simulink model "PV_BESS_EMS_PRICE"  (R2026a)
settings: Solver=FixedStepDiscrete  StopTime=86400  FixedStep=900
undefined symbols (not defined in the file): E_batt_kWh, P_batt_max_kW, P_grid_limit_kW, precharge_enable, price_aware_enable, price_low_threshold_RMB_MWh
settings Model: Creator=陈进  LastModifiedBy=陈进

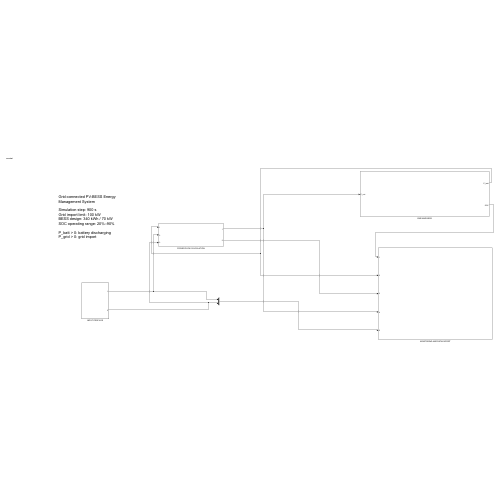
[thumbnail: Simulink's stored preview of the top-level diagram]
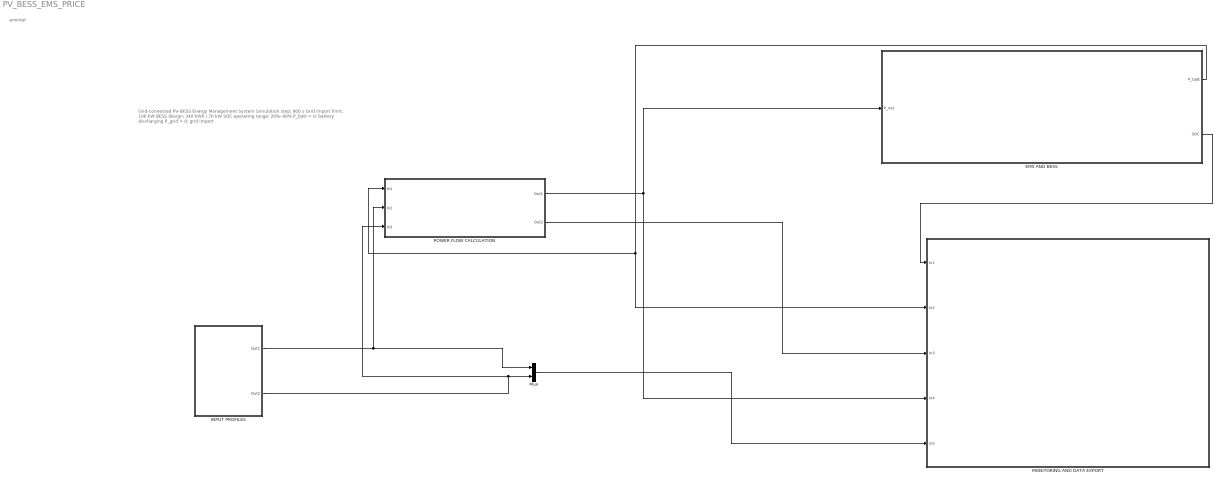
== system PV_BESS_EMS_PRICE ==
  note: Grid-connected PV-BESS Energy Management System
      |
      | Simulation step: 900 s
      | Grid import limit: 100 kW
      | BESS design: 340 kWh / 70 kW
      | SOC operating range: 20%–90%
      |
      | P_batt > 0: battery discharging
      | P_grid > 0: grid import
  note: annotat
  EMS AND BESS : Subsystem
  INPUT PROFILES : Subsystem
  MONITORING AND DATA EXPORT : Subsystem
  Mux : Mux  Inputs=2
  POWER FLOW CALCULATION : Subsystem
  wires:
  INPUT PROFILES/2(Out2) -> POWER FLOW CALCULATION/3(In3), Mux/2
  INPUT PROFILES/1(Out1) -> Mux/1, POWER FLOW CALCULATION/2(In2)
  POWER FLOW CALCULATION/1(Out1) -> MONITORING AND DATA EXPORT/4(In4), EMS AND BESS/1(P_net)
  EMS AND BESS/1(P_batt) -> POWER FLOW CALCULATION/1(In1), MONITORING AND DATA EXPORT/2(In2)
  EMS AND BESS/2(SOC) -> MONITORING AND DATA EXPORT/1(In1)
  POWER FLOW CALCULATION/2(Out2) -> MONITORING AND DATA EXPORT/3(In3)
  Mux/1 -> MONITORING AND DATA EXPORT/5(In5)

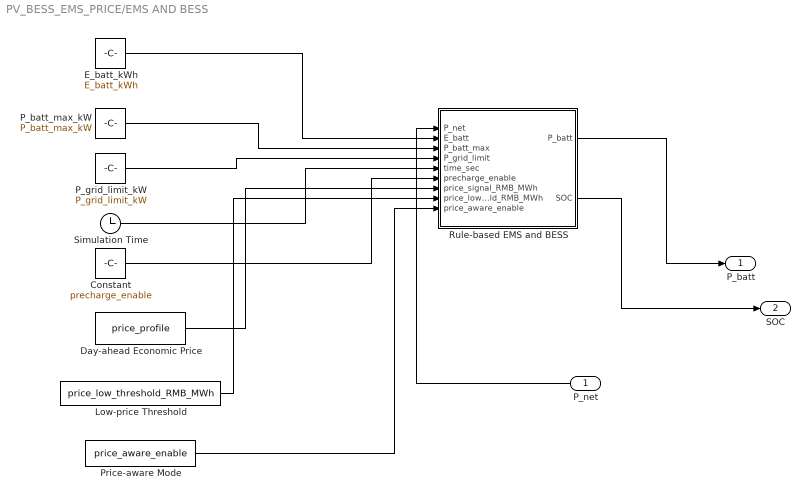
== system PV_BESS_EMS_PRICE/EMS AND BESS ==
  P_net : Inport
  Constant : Constant  Value=precharge_enable
  Day-ahead Economic Price : FromWorkspace  VariableName=price_profile
  E_batt_kWh : Constant  Value=E_batt_kWh
  Low-price Threshold : Constant  Value=price_low_threshold_RMB_MWh
  P_batt_max_kW : Constant  Value=P_batt_max_kW
  P_grid_limit_kW : Constant  Value=P_grid_limit_kW
  Price-aware Mode : Constant  Value=price_aware_enable
  Rule-based EMS and BESS : MATLAB Function  TreatAsAtomicUnit=on
  Simulation Time : Clock
  P_batt : Outport
  SOC : Outport  Port=2
  wires:
  E_batt_kWh/1 -> Rule-based EMS and BESS/2(E_batt)
  Rule-based EMS and BESS/1(P_batt) -> P_batt/1
  P_batt_max_kW/1 -> Rule-based EMS and BESS/3(P_batt_max)
  Rule-based EMS and BESS/2(SOC) -> SOC/1
  P_net/1 -> Rule-based EMS and BESS/1(P_net)
  Simulation Time/1 -> Rule-based EMS and BESS/5(time_sec)
  Constant/1 -> Rule-based EMS and BESS/6(precharge_enable)
  P_grid_limit_kW/1 -> Rule-based EMS and BESS/4(P_grid_limit)
  Day-ahead Economic Price/1 -> Rule-based EMS and BESS/7(price_signal_RMB_MWh)
  Low-price Threshold/1 -> Rule-based EMS and BESS/8(price_low_threshold_RMB_MWh)
  Price-aware Mode/1 -> Rule-based EMS and BESS/9(price_aware_enable)

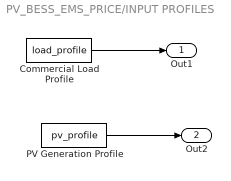
== system PV_BESS_EMS_PRICE/INPUT PROFILES ==
  Commercial Load Profile : FromWorkspace  VariableName=load_profile
  PV Generation Profile : FromWorkspace  VariableName=pv_profile
  Out1 : Outport
  Out2 : Outport  Port=2
  wires:
  PV Generation Profile/1 -> Out2/1
  Commercial Load Profile/1 -> Out1/1

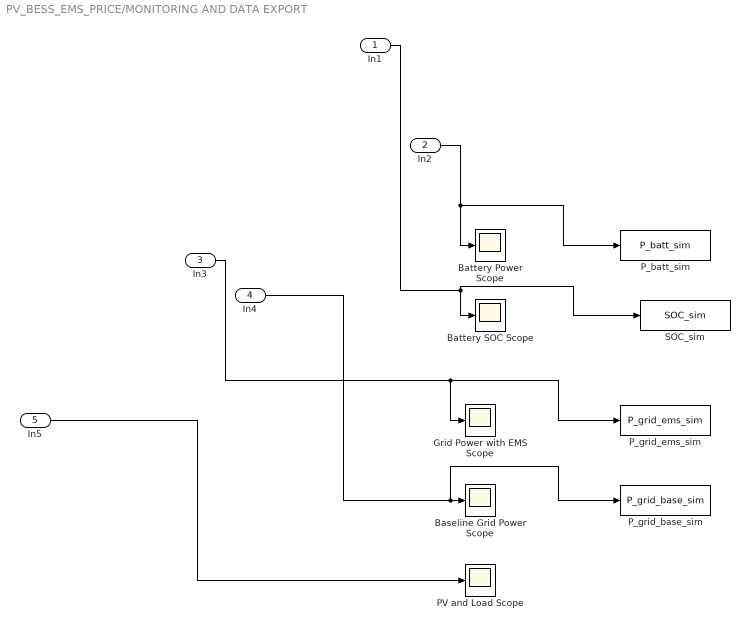
== system PV_BESS_EMS_PRICE/MONITORING AND DATA EXPORT ==
  In1 : Inport
  In2 : Inport  Port=2
  In3 : Inport  Port=3
  In4 : Inport  Port=4
  In5 : Inport  Port=5
  Baseline Grid Power Scope : Scope
      settings: ActiveDisplayYMinimum=-1  ActiveDisplayYMaximum=1
  Battery Power Scope : Scope
      settings: ActiveDisplayYMinimum=-1  ActiveDisplayYMaximum=1  DataLoggingVariableName=ScopeData4
  Battery SOC Scope : Scope
      settings: ActiveDisplayYMinimum=-1  ActiveDisplayYMaximum=1  DataLoggingVariableName=ScopeData3
  Grid Power with EMS Scope : Scope
      settings: ActiveDisplayYMinimum=-29.822290928643724  ActiveDisplayYMaximum=122.11599032135629  DataLoggingVariableName=ScopeData2
  PV and Load Scope : Scope
      settings: ActiveDisplayYMinimum=-17.499999999999996  ActiveDisplayYMaximum=157.5
  P_batt_sim : ToWorkspace  VariableName=P_batt_sim  SaveFormat=Timeseries  SampleTime=-1
  P_grid_base_sim : ToWorkspace  VariableName=P_grid_base_sim  SaveFormat=Timeseries  SampleTime=-1
  P_grid_ems_sim : ToWorkspace  VariableName=P_grid_ems_sim  SaveFormat=Timeseries  SampleTime=-1
  SOC_sim : ToWorkspace  VariableName=SOC_sim  SaveFormat=Timeseries  SampleTime=-1
  wires:
  In1/1 -> Battery SOC Scope/1, SOC_sim/1
  In4/1 -> P_grid_base_sim/1, Baseline Grid Power Scope/1
  In3/1 -> Grid Power with EMS Scope/1, P_grid_ems_sim/1
  In2/1 -> Battery Power Scope/1, P_batt_sim/1
  In5/1 -> PV and Load Scope/1

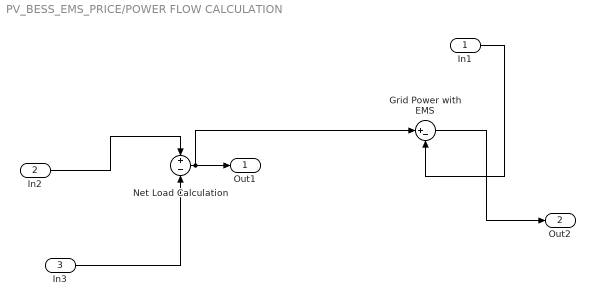
== system PV_BESS_EMS_PRICE/POWER FLOW CALCULATION ==
  In1 : Inport
  In2 : Inport  Port=2
  In3 : Inport  Port=3
  Grid Power with EMS : Sum  Inputs=|+-
  Net Load Calculation : Sum  Inputs=+-
  Out1 : Outport
  Out2 : Outport  Port=2
  wires:
  Net Load Calculation/1 -> Out1/1, Grid Power with EMS/1
  In3/1 -> Net Load Calculation/2
  In1/1 -> Grid Power with EMS/2
  In2/1 -> Net Load Calculation/1
  Grid Power with EMS/1 -> Out2/1

== matlab function PV_BESS_EMS_PRICE/EMS AND BESS/Rule-based EMS and BESS ==
  data: P_net input; P_batt output; SOC output; E_batt input; P_batt_max input; P_grid_limit input; time_sec input; precharge_enable input; price_signal_RMB_MWh input; price_low_threshold_RMB_MWh input; price_aware_enable input; SOC_initial parameter
function [P_batt, SOC] = fcn( ...
    P_net, E_batt, P_batt_max, P_grid_limit, ...
    time_sec, precharge_enable, ...
    price_signal_RMB_MWh, ...
    price_low_threshold_RMB_MWh, ...
    price_aware_enable, ...
    SOC_initial)
% Rule-based EMS with fixed-window or price-aware grid precharging
%
% P_net > 0: load demand exceeds PV generation
% P_net < 0: PV surplus is available
% P_batt > 0: battery discharging
% P_batt < 0: battery charging
% P_grid = P_net - P_batt
%
% Price-aware operation only changes grid precharging.
% PV-surplus charging and peak shaving retain their original priority.

%#codegen

%% Fixed simulation and battery parameters

dt = 900;                          % s

P_ch_max = P_batt_max;             % kW
P_dis_max = P_batt_max;            % kW

SOC_min = 0.20;
SOC_max = 0.90;

SOC_init = min(max( ...
    SOC_initial, SOC_min), SOC_max);

SOC_precharge_target = 0.90;

eta_ch = 0.95;
eta_dis = 0.95;

%% Battery state

persistent soc

if isempty(soc)
    soc = SOC_init;
end

%% Precharge-window selection

% Original validated precharge window.
is_fixed_precharge_window = ...
    (time_sec >= 0) && ...
    (time_sec < 6 * 3600);

% Check the external market-price inputs.
price_data_valid = ...
    isfinite(price_signal_RMB_MWh) && ...
    isfinite(price_low_threshold_RMB_MWh);

% Price-aware charging must occur before the evening peak.
is_low_price_before_deadline = ...
    (time_sec >= 0) && ...
    (time_sec < 17 * 3600) && ...
    price_data_valid && ...
    (price_signal_RMB_MWh <= ...
    price_low_threshold_RMB_MWh);

% Select operating mode.
if price_aware_enable > 0.5

    if price_data_valid
        is_precharge_window = ...
            is_low_price_before_deadline;
    else
        % Safe fallback if the price signal is unavailable.
        is_precharge_window = ...
            is_fixed_precharge_window;
    end

else
    is_precharge_window = ...
        is_fixed_precharge_window;
end

%% EMS decision logic

P_batt = 0;

% Rule 1: use PV surplus to charge the battery.
% This rule is never blocked by electricity price.
if P_net < 0 && soc < SOC_max

    P_charge_soc_max = ...
        (SOC_max - soc) * E_batt * 3600 ...
        / (eta_ch * dt);

    P_batt = -min( ...
        -P_net, ...
        min(P_ch_max, P_charge_soc_max));

% Rule 2: grid precharging.
% The price condition only enables the request.
% Grid headroom, SOC and power limits still apply.
elseif precharge_enable > 0.5 ...
        && is_precharge_window ...
        && soc < SOC_precharge_target ...
        && P_net < P_grid_limit

    P_charge_soc_max = ...
        (SOC_precharge_target - soc) ...
        * E_batt * 3600 ...
        / (eta_ch * dt);

    P_grid_headroom = ...
        max(P_grid_limit - P_net, 0);

    P_batt = -min( ...
        P_ch_max, ...
        min(P_charge_soc_max, ...
        P_grid_headroom));

% Rule 3: discharge for peak shaving.
elseif P_net > P_grid_limit ...
        && soc > SOC_min

    P_discharge_soc_max = ...
        (soc - SOC_min) ...
        * E_batt * 3600 ...
        * eta_dis / dt;

    P_batt = min( ...
        P_net - P_grid_limit, ...
        min(P_dis_max, ...
        P_discharge_soc_max));
end

%% SOC update

if P_batt < 0

    soc = soc + ...
        (-P_batt) * eta_ch * dt ...
        / (E_batt * 3600);

elseif P_batt > 0

    soc = soc - ...
        P_batt * dt ...
        / (eta_dis * E_batt * 3600);
end

%% Numerical safety limits

soc = min(max(soc, SOC_min), SOC_max);

SOC = soc;
